simulink model "model3"  (R2025b)
settings: Solver=VariableStepAuto  StartTime=0.0  StopTime=10.0  RelTol=1e-3
settings Model: Creator=emin  LastModifiedBy=emin

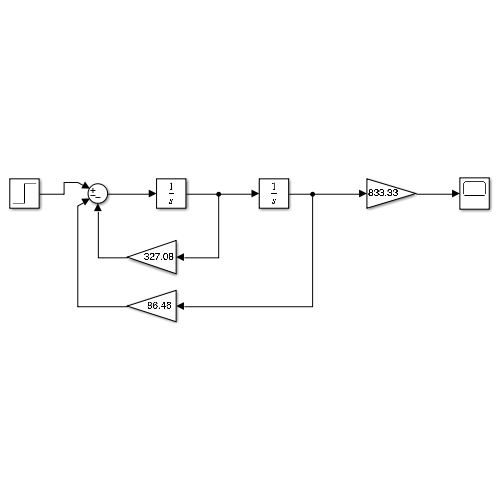
[thumbnail: Simulink's stored preview of the top-level diagram]
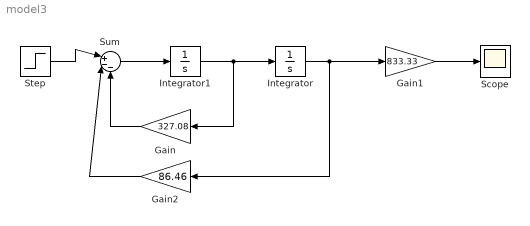
== system model3 ==
  Gain : Gain  Gain=327.08
  Gain1 : Gain  Gain=833.33
  Gain2 : Gain  Gain=86.46
  Integrator : Integrator
  Integrator1 : Integrator
  Scope : Scope
  Step : Step  SampleTime=0
  Sum : Sum  Inputs=|+--
  wires:
  Step/1 -> Sum/1
  Sum/1 -> Integrator1/1
  Integrator1/1 -> Gain/1, Integrator/1
  Integrator/1 -> Gain1/1, Gain2/1
  Gain2/1 -> Sum/2
  Gain/1 -> Sum/3
  Gain1/1 -> Scope/1
